simulink library "PID_Lib"  (R2022b)
settings: Solver=VariableStepAuto  StartTime=0.0  StopTime=10.0  RelTol=1e-3
undefined symbols (not defined in the file): DiscIntNeverNeededParam
libraries: simulink x2
settings Model: Creator=user  LastModifiedBy=user

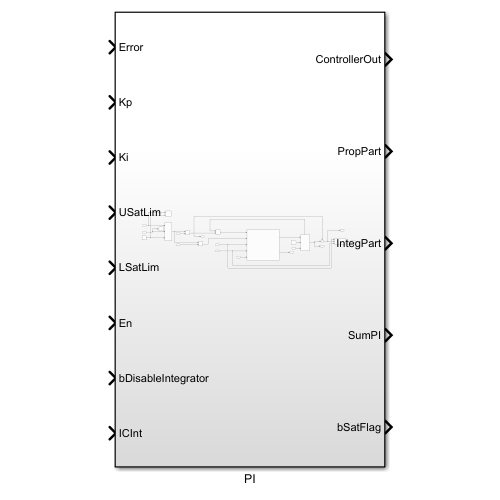
[thumbnail: Simulink's stored preview of the top-level diagram]
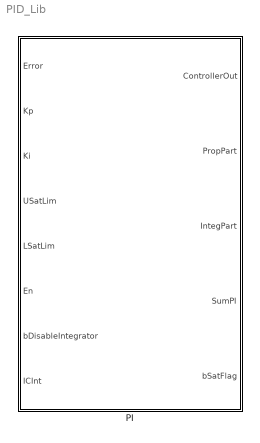
== system PID_Lib ==
  PI : Subsystem

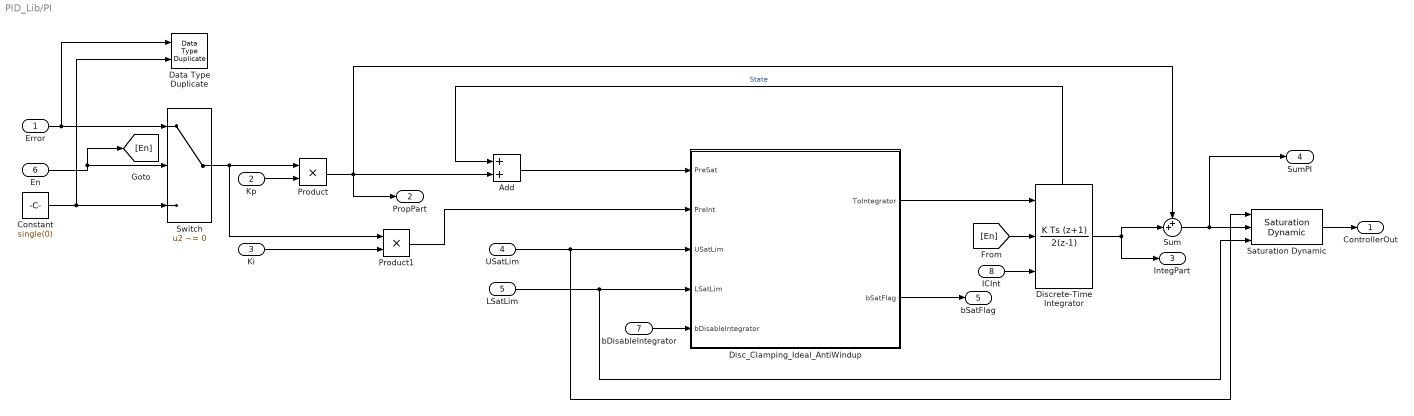
== system PID_Lib/PI ==
  Error : Inport
  Kp : Inport  Port=2
  Ki : Inport  Port=3
  USatLim : Inport  Port=4
  LSatLim : Inport  Port=5
  En : Inport  Port=6
  bDisableIntegrator : Inport  Port=7
  ICInt : Inport  Port=8
  Add : Sum  OutDataTypeStr=Inherit: Inherit via back propagation
  Constant : Constant  Value=single(0)
  Data Type Duplicate : DataTypeDuplicate
  Disc_Clamping_Ideal_AntiWindup : Subsystem
  Discrete-Time Integrator : DiscreteIntegrator  IntegratorMethod=Integration: Trapezoidal  ExternalReset=either  InitialConditionSource=external  SampleTime=-1  OutDataTypeStr=Inherit: Inherit via back propagation  ShowStatePort=on  ICPrevOutput=DiscIntNeverNeededParam  ICPrevScaledInput=DiscIntNeverNeededParam
      settings: AttributesFormatString=|
      | %<SampleTime>
      | %<IntegratorMethod>
      | %<ExternalReset>
  Product : Product  OutDataTypeStr=Inherit: Inherit via back propagation
  Product1 : Product  OutDataTypeStr=Inherit: Inherit via back propagation
  Saturation Dynamic : simulink/Discontinuities/Saturation Dynamic  OutMin=[]  OutMax=[]  OutDataTypeStr=Inherit: Same as second input  OutDataType=fixdt(1, 16)  OutScaling=2^-10  DoSatur=off
  Sum : Sum  Inputs=++|  OutDataTypeStr=Inherit: Inherit via back propagation
  Switch : Switch  Criteria=u2 ~= 0  OutDataTypeStr=Inherit: Inherit via back propagation  SaturateOnIntegerOverflow=off  InputSameDT=off
  ControllerOut : Outport
  PropPart : Outport  Port=2
  IntegPart : Outport  Port=3
  SumPI : Outport  Port=4
  bSatFlag : Outport  Port=5
  wires:
  Constant/1 -> Data Type Duplicate/2, Switch/3
  Product1/1 -> Disc_Clamping_Ideal_AntiWindup/2(PreInt)
  Disc_Clamping_Ideal_AntiWindup/2(bSatFlag) -> bSatFlag/1
  Sum/1 -> SumPI/1, Saturation Dynamic/2
  Switch/1 -> Product1/1, Product/1
  Discrete-Time Integrator/1 -> Sum/2, IntegPart/1
  LSatLim/1 -> Disc_Clamping_Ideal_AntiWindup/4(LSatLim), Saturation Dynamic/3
  Add/1 -> Disc_Clamping_Ideal_AntiWindup/1(PreSat)
  Error/1 -> Data Type Duplicate/1, Switch/1
  Product/1 -> PropPart/1, Sum/1, Add/2
  USatLim/1 -> Disc_Clamping_Ideal_AntiWindup/3(USatLim), Saturation Dynamic/1
  Discrete-Time Integrator/State -> Add/1  "State"
  En/1 -> Switch/2, [En]
  Kp/1 -> Product/2
  Ki/1 -> Product1/2
  [En] -> Discrete-Time Integrator/2
  Disc_Clamping_Ideal_AntiWindup/1(ToIntegrator) -> Discrete-Time Integrator/1
  bDisableIntegrator/1 -> Disc_Clamping_Ideal_AntiWindup/5(bDisableIntegrator)
  Saturation Dynamic/1 -> ControllerOut/1
  ICInt/1 -> Discrete-Time Integrator/3

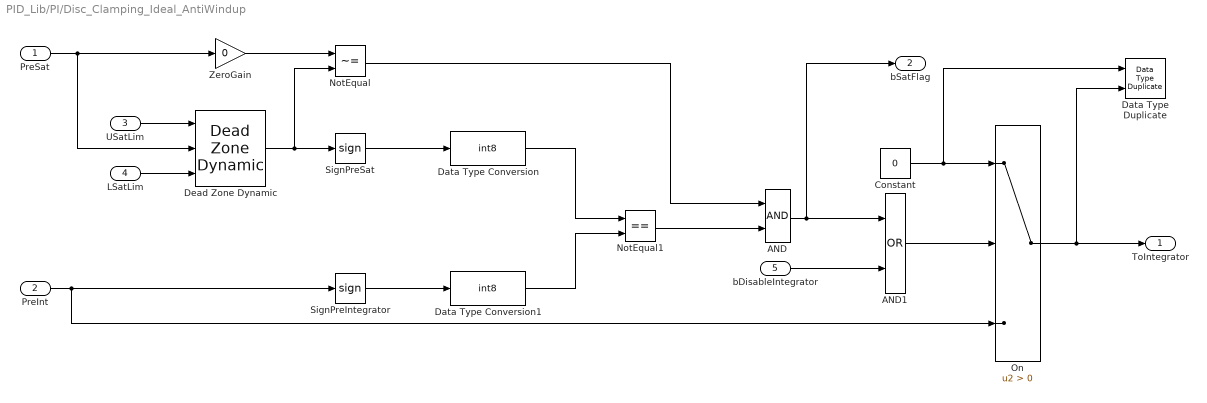
== system PID_Lib/PI/Disc_Clamping_Ideal_AntiWindup ==
  PreSat : Inport
  PreInt : Inport  Port=2
  USatLim : Inport  Port=3
  LSatLim : Inport  Port=4
  bDisableIntegrator : Inport  Port=5
  AND : Logic  AllPortsSameDT=off  OutDataTypeStr=boolean
  AND1 : Logic  Operator=OR  AllPortsSameDT=off  OutDataTypeStr=boolean
  Constant : Constant  Value=0
  Data Type Duplicate : DataTypeDuplicate
  Data Type Conversion : DataTypeConversion  OutDataTypeStr=int8  SaturateOnIntegerOverflow=off  RndMeth=Floor
  Data Type Conversion1 : DataTypeConversion  OutDataTypeStr=int8  SaturateOnIntegerOverflow=off  RndMeth=Floor
  Dead Zone Dynamic : simulink/Discontinuities/Dead Zone Dynamic
  NotEqual : RelationalOperator  Operator=~=  OutDataTypeStr=boolean  RndMeth=Simplest  InputSameDT=off
  NotEqual1 : RelationalOperator  Operator===  OutDataTypeStr=boolean  RndMeth=Simplest  InputSameDT=off
  On : Switch  Criteria=u2 > Threshold  SaturateOnIntegerOverflow=off  InputSameDT=off
  SignPreIntegrator : Signum
  SignPreSat : Signum
  ZeroGain : Gain  Gain=0
  ToIntegrator : Outport
  bSatFlag : Outport  Port=2
  wires:
  AND/1 -> bSatFlag/1, AND1/1
  Dead Zone Dynamic/1 -> NotEqual/2, SignPreSat/1
  Constant/1 -> Data Type Duplicate/1, On/1
  PreInt/1 -> On/3, SignPreIntegrator/1
  bDisableIntegrator/1 -> AND1/2
  NotEqual1/1 -> AND/2
  SignPreIntegrator/1 -> Data Type Conversion1/1
  Data Type Conversion1/1 -> NotEqual1/2
  On/1 -> ToIntegrator/1, Data Type Duplicate/2
  PreSat/1 -> ZeroGain/1, Dead Zone Dynamic/2
  AND1/1 -> On/2
  NotEqual/1 -> AND/1
  SignPreSat/1 -> Data Type Conversion/1
  Data Type Conversion/1 -> NotEqual1/1
  USatLim/1 -> Dead Zone Dynamic/1
  ZeroGain/1 -> NotEqual/1
  LSatLim/1 -> Dead Zone Dynamic/3
